simulink model "ecu_underg"  (R2026a)
settings: Solver=FixedStepDiscrete  StopTime=10  FixedStep=0.001  SampleTimeConstraint=STIndependent
Description:
  | Underspeed warning. Source of truth for firmware/gen/ecu_underg.
settings Model: Creator=jj1001000  LastModifiedBy=jj1001000
settings OptimizationCC: DefaultUnderspecifiedDataType=single
settings DebuggingCC: ParameterPrecisionLossMsg=none
settings HardwareCC: ProdLargestAtomicInteger=Long  ProdLargestAtomicFloat=Double  ProdHWDeviceType=ARM Compatible->ARM Cortex-M
settings RTWCC: SystemTargetFile=ert.tlc  GenCodeOnly=on  Description=Embedded Coder
settings ERTTargetCC: UtilityFuncGeneration=Shared location  IncludeMdlTerminateFcn=off  CodeInterfacePackaging=Reusable function  SupportNonFinite=off

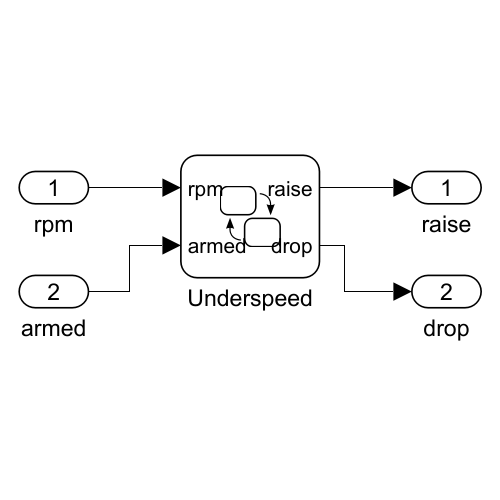
[thumbnail: Simulink's stored preview of the top-level diagram]
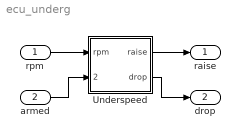
== system ecu_underg ==
  rpm : Inport  OutDataTypeStr=single
  armed : Inport  Port=2  OutDataTypeStr=uint8
  Underspeed : Stateflow chart  TreatAsAtomicUnit=on
  raise : Outport  OutDataTypeStr=uint8
  drop : Outport  Port=2  OutDataTypeStr=uint8
  wires:
  rpm/1 -> Underspeed/1(rpm)
  Underspeed/2(drop) -> drop/1
  armed/1 -> Underspeed/2(armed)
  Underspeed/1(raise) -> raise/1

== stateflow chart ecu_underg/Underspeed ==
  settings: updateMethod=DISCRETE  executeAtInitialization=1
  state DISARMED
    entry: raise = uint8(0); drop = uint8(1);
  state ARMED
    state MID
      entry: raise = uint8(0); drop = uint8(0);
    state LOW_COUNT
      entry: raise = uint8(0); drop = uint8(0);
      during: n = n + 1;
    state HIGH_COUNT
      entry: raise = uint8(0); drop = uint8(0);
      during: n = n + 1;
    state LOW
      entry: raise = uint8(1); drop = uint8(0);
    state HIGH
      entry: raise = uint8(0); drop = uint8(1);
    (default) -> MID
    LOW_COUNT -> MID [order 2] : [rpm >= single(1350)]
    HIGH_COUNT -> MID [order 2] : [rpm <= single(1400)]
    MID -> LOW_COUNT [order 1] : [rpm < single(1350)]{n = uint16(1);}
    MID -> HIGH_COUNT [order 2] : [rpm > single(1400)]{n = uint16(1);}
    LOW -> MID [order 2] : [rpm >= single(1350)]
    HIGH -> MID [order 2] : [rpm <= single(1400)]
    LOW_COUNT -> HIGH_COUNT [order 1] : [rpm > single(1400)]{n = uint16(1);}
    HIGH_COUNT -> LOW_COUNT [order 1] : [rpm < single(1350)]{n = uint16(1);}
    LOW_COUNT -> LOW [order 3] : [n + 1 >= uint16(3000)]
    HIGH -> LOW_COUNT [order 1] : [rpm < single(1350)]{n = uint16(1);}
    LOW -> HIGH_COUNT [order 1] : [rpm > single(1400)]{n = uint16(1);}
    HIGH_COUNT -> HIGH [order 3] : [n + 1 >= uint16(1000)]
  (default) -> DISARMED : {n = uint16(0);}
  DISARMED -> HIGH_COUNT [order 2] : [armed ~= 0 && rpm > single(1400)]{n = uint16(1);}
  DISARMED -> MID [order 3] : [armed ~= 0]
  ARMED -> DISARMED : [armed == 0]
  DISARMED -> LOW_COUNT [order 1] : [armed ~= 0 && rpm < single(1350)]{n = uint16(1);}
  data: rpm input single; armed input uint8; raise output uint8; drop output uint8; n local uint16
